simulink model "axis_rocket_stablilty_model"  (R2026b)
settings: Solver=VariableStepAuto
values from neighbouring files (symbols this model uses):
  den_P = [J_v, b, 0]    [Model_rocket_stablizer.m]    (also in Model_rocket_stablizer_revised.m)
  Kd = 350.6    [Model_rocket_stablizer.m]    (also in Model_rocket_stablizer_revised.m = 73.18; build_rocket_roll_model.m = 73.18;'])
  Ki = 2953.68    [Model_rocket_stablizer.m]    (also in Model_rocket_stablizer_revised.m = 616.37; build_rocket_roll_model.m = 616.37)
  Kp = 1772.21    [Model_rocket_stablizer.m]    (also in Model_rocket_stablizer_revised.m = 369.82)
  num_P = [J_w]    [Model_rocket_stablizer.m]    (also in Model_rocket_stablizer_revised.m)
settings Model: Creator=Nirmal Krishna P  LastModifiedBy=Nirmal Krishna P

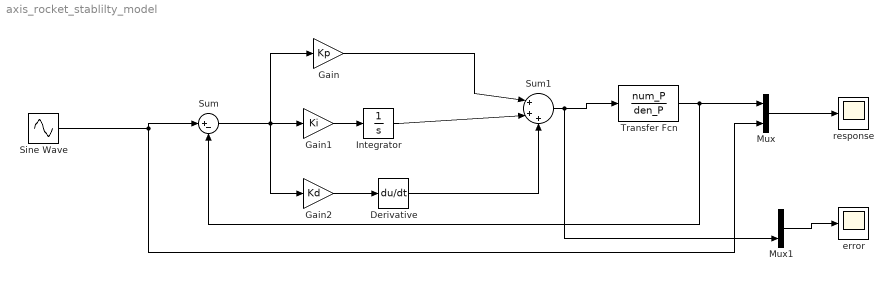
== system axis_rocket_stablilty_model ==
  Derivative : Derivative
  Gain : Gain  Gain=Kp
  Gain1 : Gain  Gain=Ki
  Gain2 : Gain  Gain=Kd
  Integrator : Integrator
  Mux : Mux  Inputs=2
  Mux1 : Mux  Inputs=2
  Sine Wave : Sin  SampleTime=0
  Sum : Sum  Inputs=|+-
  Sum1 : Sum  Inputs=|+++
  Transfer Fcn : TransferFcn  Numerator=num_P  Denominator=den_P
  error : Scope
      settings: ActiveDisplayYMinimum=-864.73950632831918  ActiveDisplayYMaximum=1130.0754170308212
  response : Scope
      settings: ActiveDisplayYMinimum=-0.94106341191606036  ActiveDisplayYMaximum=1.1876641416386398
  wires:
  Sum/1 -> Gain/1, Gain2/1, Gain1/1
  Gain1/1 -> Integrator/1
  Gain2/1 -> Derivative/1
  Derivative/1 -> Sum1/3
  Integrator/1 -> Sum1/2
  Gain/1 -> Sum1/1
  Sum1/1 -> Mux1/2, Transfer Fcn/1
  Mux/1 -> response/1
  Sine Wave/1 -> Mux/2, Sum/1
  Mux1/1 -> error/1
  Transfer Fcn/1 -> Sum/2, Mux/1
